simulink model "audit_uq_component"  (R2025a)
settings: Solver=FixedStepDiscrete  StartTime=0.0  StopTime=0  FixedStep=1  RelTol=1e-3
model workspace (MAT data in the model file):
  mMaxCurrent = 0.99
settings Model: Creator=alexey  LastModifiedBy=alexey

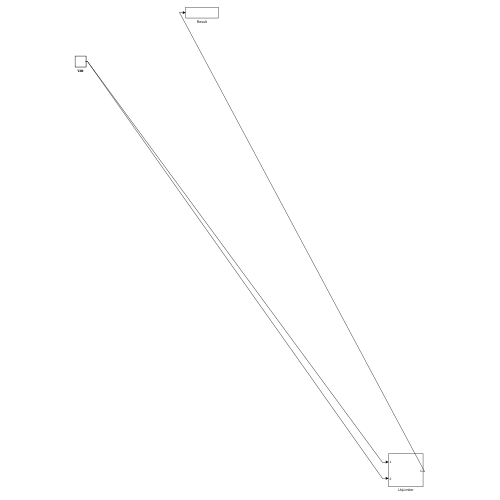
[thumbnail: Simulink's stored preview of the top-level diagram]
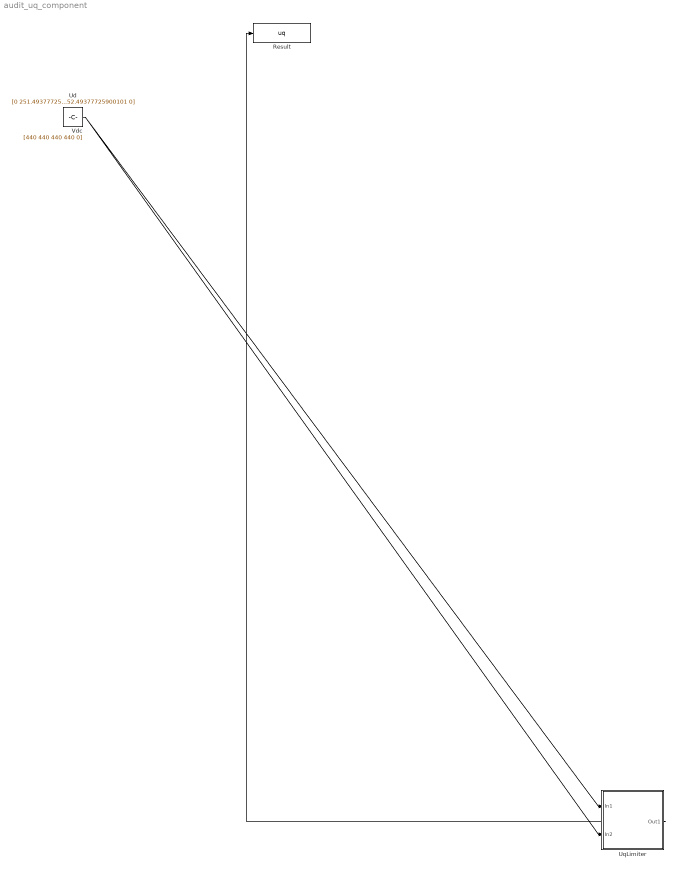
== system audit_uq_component ==
  Result : ToWorkspace  VariableName=uq  SampleTime=-1
  Ud : Constant  Value=[0 251.49377725900101 -251.49377725900101 252.49377725900101 0]
  UqLimiter : Subsystem
  Vdc : Constant  Value=[440 440 440 440 0]
  wires:
  Ud/1 -> UqLimiter/1(In1)
  Vdc/1 -> UqLimiter/2(In2)
  UqLimiter/1(Out1) -> Result/1

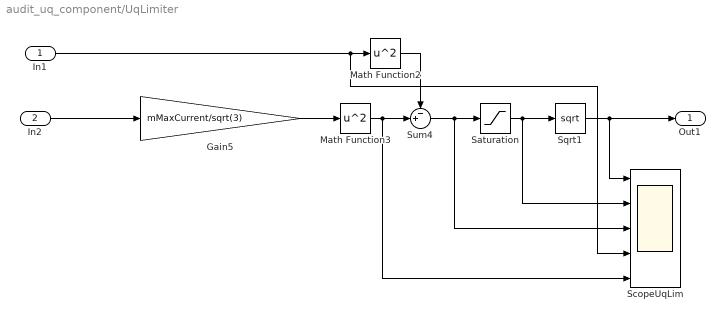
== system audit_uq_component/UqLimiter ==
  In1 : Inport
  In2 : Inport  Port=2
  Gain5 : Gain  Gain=mMaxCurrent/sqrt(3)
  Math Function2 : Math  Operator=square
  Math Function3 : Math  Operator=square
  Saturation : Saturate  UpperLimit=inf  LowerLimit=0.001
  ScopeUqLim : Scope  NumInputPorts=5
      settings: ActiveDisplayYMinimum=149.70176366248859  ActiveDisplayYMaximum=275.51811800976793  DataLoggingVariableName=ScopeData5
  Sqrt1 : Sqrt
  Sum4 : Sum  Inputs=-+|
  Out1 : Outport
  wires:
  Saturation/1 -> ScopeUqLim/2, Sqrt1/1
  Math Function3/1 -> ScopeUqLim/5, Sum4/2
  Gain5/1 -> Math Function3/1
  In2/1 -> Gain5/1
  Math Function2/1 -> Sum4/1
  Sum4/1 -> ScopeUqLim/3, Saturation/1
  Sqrt1/1 -> ScopeUqLim/1, Out1/1
  In1/1 -> ScopeUqLim/4, Math Function2/1
